simulink model "test_thd"  (R2026a)
settings: Solver=VariableStepAuto  StopTime=1
values from neighbouring files (symbols this model uses):
  glb_time = timing_setup(fpwm_afe, trgo_afe, fpwm_inv, trgo_inv, fpwm_single_phase_inv, trgo_single_phase_inv, fpwm_dab, trgo_dab,      fpwm_psfbc, trgo_psfbc, fpwm_isop_rail, trgo_isop_rail, fpwm_cllc, trgo_cllc, t_measure, tc_factor, tc_decimation, delay_pwm, dead_time_afe,      dead_time_inv, dead_time_single_phase_inv, dead_time_dab, dead_time_psfbc, dead_time_isop_rail, dead_time_cllc)    [init_model_legacy.m]
settings Model: Creator=dbagn  LastModifiedBy=dbagn

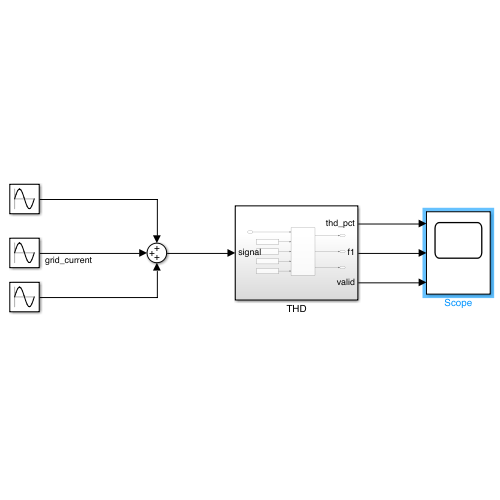
[thumbnail: Simulink's stored preview of the top-level diagram]
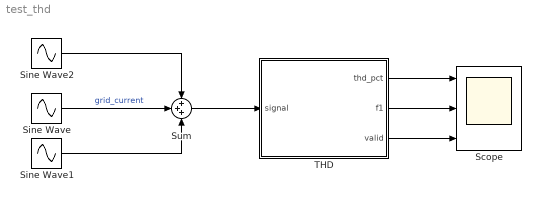
== system test_thd ==
  Scope : Scope  NumInputPorts=3
      settings: ActiveDisplayYMinimum=-3.5355339059327444  ActiveDisplayYMaximum=31.819805153394707
  Sine Wave : Sin  Frequency=2*pi*50  SampleTime=0
  Sine Wave1 : Sin  Amplitude=0.2  Frequency=2*pi*50*2  SampleTime=0
  Sine Wave2 : Sin  Amplitude=0.2  Frequency=2*pi*50*4  SampleTime=0
  Sum : Sum  Inputs=+++
  THD : Subsystem
  wires:
  THD/1(thd_pct) -> Scope/1
  THD/2(f1) -> Scope/2
  THD/3(valid) -> Scope/3
  Sum/1 -> THD/1(signal)
  Sine Wave/1 -> Sum/2  "grid_current"
  Sine Wave1/1 -> Sum/3
  Sine Wave2/1 -> Sum/1

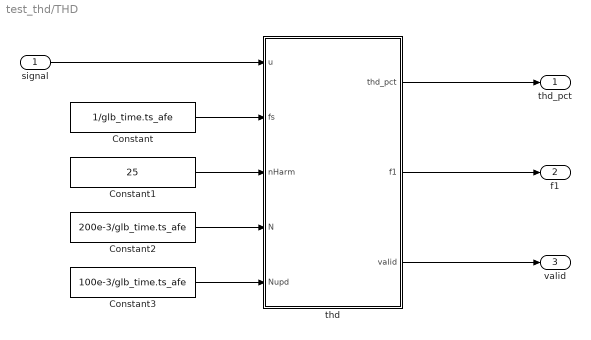
== system test_thd/THD ==
  signal : Inport
  Constant : Constant  Value=1/glb_time.ts_afe
  Constant1 : Constant  Value=25
  Constant2 : Constant  Value=200e-3/glb_time.ts_afe
  Constant3 : Constant  Value=100e-3/glb_time.ts_afe
  thd : MATLAB Function  TreatAsAtomicUnit=on  SystemSampleTime=glb_time.ts_afe
  thd_pct : Outport
  f1 : Outport  Port=2
  valid : Outport  Port=3
  wires:
  Constant3/1 -> thd/5(Nupd)
  signal/1 -> thd/1(u)
  Constant2/1 -> thd/4(N)
  thd/2(f1) -> f1/1
  thd/1(thd_pct) -> thd_pct/1
  Constant1/1 -> thd/3(nHarm)
  Constant/1 -> thd/2(fs)
  thd/3(valid) -> valid/1

== matlab function test_thd/THD/thd ==
  data: u input; thd_pct output; f1 output; valid output; fs input; nHarm input; N input; Nupd input
function [thd_pct, f1, valid] = thd_online(u, fs, nHarm, N, Nupd)
%#codegen
% THD online con buffer circolare interno, per MATLAB Function block.
%
%   u     : ingresso scalare (un campione per passo, a frequenza fs)
%   fs    : frequenza di campionamento [Hz]
%   nHarm : n. di armoniche del THD (es. 40)
%   N     : lunghezza del buffer in campioni (es. 20 periodi di f1)
%   Nupd  : ogni quanti campioni ricalcolare il THD (es. N/4)
%
%   thd_pct : THD in %, tenuto costante tra un ricalcolo e l'altro
%   f1      : fondamentale stimata [Hz]
%   valid   : false finche' il buffer non e' pieno la prima volta

persistent buf k nfill ncnt thd_p f1_p
if isempty(buf)
    buf   = zeros(N,1);
    k     = 1;          % indice di scrittura circolare
    nfill = 0;          % campioni acquisiti (satura a N)
    ncnt  = 0;          % contatore per il ricalcolo
    thd_p = 0;
    f1_p  = 0;
end

% --- scrittura nel buffer circolare ----------------------------------
buf(k) = u;
k = k + 1;
if k > N
    k = 1;
end
if nfill < N
    nfill = nfill + 1;
end
ncnt = ncnt + 1;

% --- ricalcolo: a buffer pieno, ogni Nupd campioni -------------------
if nfill >= N && ncnt >= Nupd
    ncnt = 0;
    % riordino cronologico (dal campione piu' vecchio al piu' recente),
    % a dimensione fissa: codegen-safe
    x = zeros(N,1);
    for i = 1:N
        j = k + i - 1;
        if j > N
            j = j - N;
        end
        x(i) = buf(j);
    end
    [thd_p, f1_p] = local_thd(x, fs, nHarm);
end

thd_pct = thd_p;
f1      = f1_p;
valid   = (nfill >= N);
end

% =====================================================================
function [thd_pct, f1] = local_thd(x, fs, nHarm)
% THD su un frame di N campioni (finestra di Hann + somma in energia)

x = x - mean(x);
N = numel(x);

n = (0:N-1).';
w = 0.5*(1 - cos(2*pi*n/N));

X   = fft(x .* w);
mag = abs(X(1:floor(N/2))) * 2/sum(w);
Nb  = numel(mag);

[~, k1] = max(mag(4:end));
k1 = k1 + 3;

d = 0;
if k1 > 1 && k1 < Nb
    den = 2*(2*mag(k1) - mag(k1+1) - mag(k1-1));
    if den ~= 0
        d = (mag(k1+1) - mag(k1-1))/den;
    end
end
f1 = (k1 - 1 + d)*fs/N;

nb = 3;
Vh = zeros(nHarm,1);
for h = 1:nHarm
    kh = round(h*(k1 - 1 + d)) + 1;
    if kh + nb > Nb
        break                          % armoniche oltre Nyquist: restano 0
    end
    lo = max(kh - 5, 2);
    hi = min(kh + 5, Nb - nb);
    [~, km] = max(mag(lo:hi));
    kp = lo + km - 1;
    Vh(h) = sqrt(sum(mag(kp-nb:kp+nb).^2)/1.5);
end

thd_pct = sqrt(sum(Vh(2:end).^2)) / max(Vh(1), eps) * 100;
end
